simulink model "demoWaveElevation"  (R2024a)
settings: Solver=ode3  StartTime=0.0  StopTime=100  FixedStep=.1  RelTol=1e-3  EnableMultiTasking=on
libraries: mssSimulink x2
settings Model: Creator=tristan  LastModifiedBy=thor
settings SolverCC: AlgebraicLoopSolver=TrustRegion
settings DataIOCC: LimitDataPoints=on  SaveFormat=Array  SignalLoggingSaveFormat=ModelDataLogs  ReturnWorkspaceOutputs=off
settings OptimizationCC: InitFltsAndDblsToZero=on  LifeSpan=inf
settings DebuggingCC: SaveWithParameterizedLinksMsg=none  UnderspecifiedInitializationDetection=Classic  MergeDetectMultiDrivingBlocksExec=none  SignalResolutionControl=TryResolveAllWithWarning  SolverPrmCheckMsg=warning  FcnCallInpInsideContextMsg=warning  UnconnectedInputMsg=warning  UnconnectedOutputMsg=warning  UnconnectedLineMsg=warning  SFUnexpectedBacktrackingDiag=warning  SFNoUnconditionalDefaultTransitionDiag=warning  SFExecutionAtInitializationDiag=none  ArithmeticOperatorsInVariantConditions=warning
settings HardwareCC: ProdBitPerPointer=32  ProdBitPerSizeT=32  ProdBitPerPtrDiffT=32  ProdLargestAtomicFloat=None  ProdIntDivRoundTo=Undefined  ProdEndianess=Unspecified  ProdWordSize=32  ProdHWDeviceType=32-bit Generic
settings ModelReferenceCC: EnableRefExpFcnMdlSchedulingChecks=on  PropagateSignalLabelsOutOfModel=off
settings RTWCC: GPUComputeCapability=3.5  DLArmComputeVersion=19.05
settings CodeAppCC: StateflowObjectComments=on
settings GRTTargetCC: TargetFcnLib=ansi_tfl_tmw.mat  TargetLangStandard=C89/C90 (ANSI)  CombineOutputUpdateFcns=off  GRTInterface=on
settings ConfigComp: CovMetricSettings=dw  CovSaveCumulativeToWorkspaceVar=on  CovSaveSingleToWorkspaceVar=on

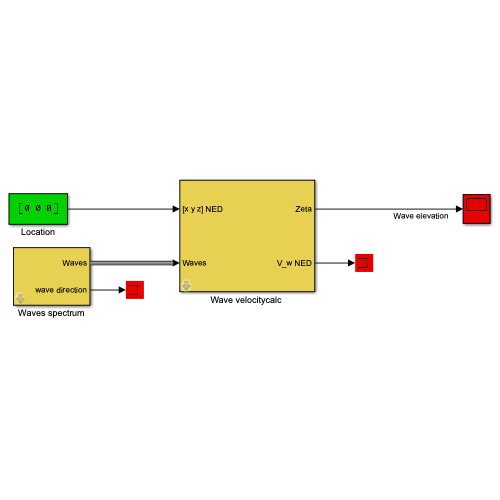
[thumbnail: Simulink's stored preview of the top-level diagram]
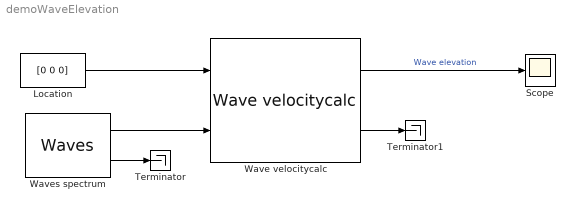
== system demoWaveElevation ==
  Location : Constant  Value=[0 0 0]
  Scope : Scope
  Terminator : Terminator
  Terminator1 : Terminator
  "Wave velocitycalc " : mssSimulink/Environment/Waves/Wave velocitycalc
  Waves spectrum : mssSimulink/Environment/Waves/Waves  spectrum_type=ITTC  disp_flag=on  plot_spectrum=on  plot_realization=on  hs=0.8  omega_peak=0  psi_mean=0  gamma=-1  spread=2  depth=inf  nfreq=20  ndir=10  energylim=0.005  freq_cutoff=3  dir_cutoff=0  rand_seed=123  rand_freq=on  rand_dir=on  Zeta_a=0  Omega=0  Phase=0  Wavenum=0  Psi=0
  wires:
  Waves spectrum/1 -> "Wave velocitycalc "/2
  Location/1 -> "Wave velocitycalc "/1
  "Wave velocitycalc "/1 -> Scope/1  "Wave elevation"
  "Wave velocitycalc "/2 -> Terminator1/1
  Waves spectrum/2 -> Terminator/1
